simulink model "CurrentSensor"  (R2026b)
settings: Solver=VariableStepAuto
values from neighbouring files (symbols this model uses):
  Cur_ADCMax = 1023    [DCMotorParams.m]
  Cur_Dir = -1    [DCMotorParams.m]
  Cur_LPF_Den = [1, Cur_LPF_a - 1]    [DCMotorParams.m]
  Cur_LPF_Num = Cur_LPF_a    (= 0.166666666667)    [DCMotorParams.m]
  Cur_OffsetV = 2.5643    [DCMotorParams.m]
  Cur_Sens = 0.185    [DCMotorParams.m]
  Cur_VRef = 5.0    (= 5)    [DCMotorParams.m]
  Ts = 0.01    [DCMotorParams.m]
libraries: arduinolib x1
settings Model: Creator=bence  LastModifiedBy=bence

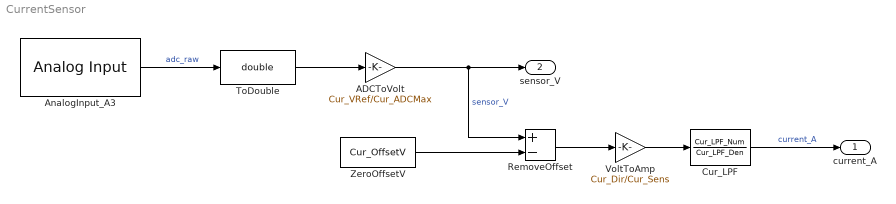
== system CurrentSensor ==
  ADCToVolt : Gain  Gain=Cur_VRef/Cur_ADCMax
  AnalogInput_A3 : arduinolib/Analog Input  pinNumber=3  ReadResultsOnly=off  ConversionTriggerSource=Software  ExternalTriggerType=uint32( 0 )  OutputDataType=uint16  EnableConversionCompleteNotify=off  EnableOuputStatus=off  SampleTime=Ts  blockPlatform=arduino
  Cur_LPF : DiscreteTransferFcn  Numerator=Cur_LPF_Num  Denominator=Cur_LPF_Den  SampleTime=Ts
  RemoveOffset : Sum  Inputs=+-
  ToDouble : DataTypeConversion  OutDataTypeStr=double  SaturateOnIntegerOverflow=off  RndMeth=Floor
  VoltToAmp : Gain  Gain=Cur_Dir/Cur_Sens
  ZeroOffsetV : Constant  Value=Cur_OffsetV
  current_A : Outport
  sensor_V : Outport  Port=2
  wires:
  Cur_LPF/1 -> current_A/1  "current_A"
  VoltToAmp/1 -> Cur_LPF/1
  RemoveOffset/1 -> VoltToAmp/1
  ZeroOffsetV/1 -> RemoveOffset/2
  ADCToVolt/1 -> RemoveOffset/1, sensor_V/1  "sensor_V"
  ToDouble/1 -> ADCToVolt/1
  AnalogInput_A3/1 -> ToDouble/1  "adc_raw"
